simulink model "pmsm_id_bench"  (R2024b)
settings: Solver=ode4  StartTime=0.0  StopTime=bench.StopTime  FixedStep=bench.SolverStep  RelTol=1e-3
model workspace (MAT data in the model file):
  bench.Rs = 0.7
  bench.Ld = 0.004
  bench.Lq = 0.006
  bench.Flux = 0.03
  bench.VoltageDrop = 0.35
  bench.ResistanceDrop = 0.03
  bench.ZeroCurrent = 0.15
  bench.Phase = 0
  bench.StopTime = 0.6
  bench.SolverStep = 1e-05
  bench.SamplePeriod = 0.0001
  bench.InitialDCurrent = 0
  bench.InitialQCurrent = 0
  bench.DVoltageBias = 1.2
  bench.DVoltageAmplitude = [0.8 0.35]
  bench.DVoltageFrequency = [31 9]
  bench.QVoltageBias = 5
  bench.QVoltageAmplitude = [1.1 0.6]
  bench.QVoltageFrequency = [17 4]
  bench.SpeedBias = 160
  bench.SpeedAmplitude = 40
  bench.SpeedFrequency = 3
values from neighbouring files (symbols this model uses):
  bench = struct('Rs',0.7,'Ld',0.004,'Lq',0.006,'Flux',0.03,      'VoltageDrop',0.35,'ResistanceDrop',0.03,'ZeroCurrent',0.15,      'Phase',0,'StopTime',0.6,'SolverStep',1e-5,'SamplePeriod',1e-4,      'InitialDCurrent',0,'InitialQCurrent',0,      'DVoltageBias',1.2,'DVoltageAmplitude',[0.8,0.35],      'DVoltageFrequency',[31,9],'QVoltageBias',5,      'QVoltageAmplitude',[1.1,0.6],'QVoltageFrequency',[17,4], ...(+61 chars)    [pmsm_bench_defaults.m]    (also in pmsm_mechanical_defaults.m = struct('J',0.002,'B',0.001,'Tc',0.02,'FrictionSpeed',0.2,   ; pmsm_run_mechanical_benchmark.m = pmsm_mechanical_defaults(); pmsm_run_simulink_benchmark.m = pmsm_bench_defaults())
settings Model: Creator=lxy  LastModifiedBy=lxy
settings DataIOCC: SignalLogging=off

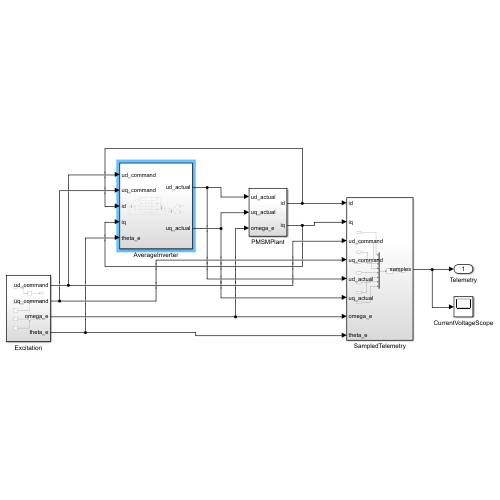
[thumbnail: Simulink's stored preview of the top-level diagram]
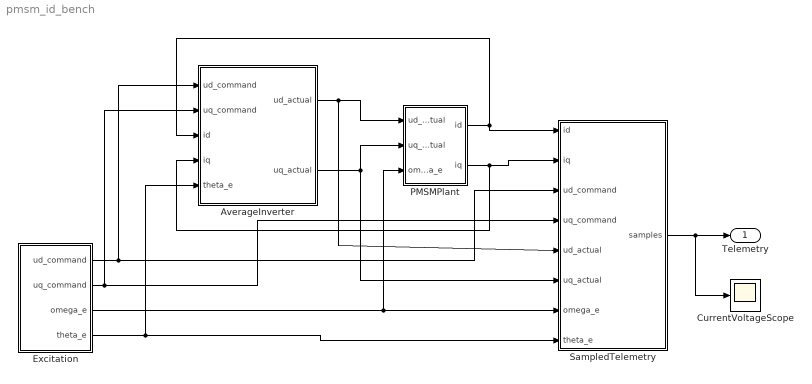
== system pmsm_id_bench ==
  AverageInverter : Subsystem
  CurrentVoltageScope : Scope
  Excitation : Subsystem
  PMSMPlant : Subsystem
  SampledTelemetry : Subsystem
  Telemetry : Outport
  wires:
  Excitation/1(ud_command) -> SampledTelemetry/3(ud_command), AverageInverter/1(ud_command)
  Excitation/2(uq_command) -> SampledTelemetry/4(uq_command), AverageInverter/2(uq_command)
  Excitation/4(theta_e) -> SampledTelemetry/8(theta_e), AverageInverter/5(theta_e)
  Excitation/3(omega_e) -> SampledTelemetry/7(omega_e), PMSMPlant/3(omega_e)
  AverageInverter/1(ud_actual) -> SampledTelemetry/5(ud_actual), PMSMPlant/1(ud_actual)
  AverageInverter/2(uq_actual) -> SampledTelemetry/6(uq_actual), PMSMPlant/2(uq_actual)
  PMSMPlant/1(id) -> SampledTelemetry/1(id), AverageInverter/3(id)
  PMSMPlant/2(iq) -> SampledTelemetry/2(iq), AverageInverter/4(iq)
  SampledTelemetry/1(samples) -> Telemetry/1, CurrentVoltageScope/1

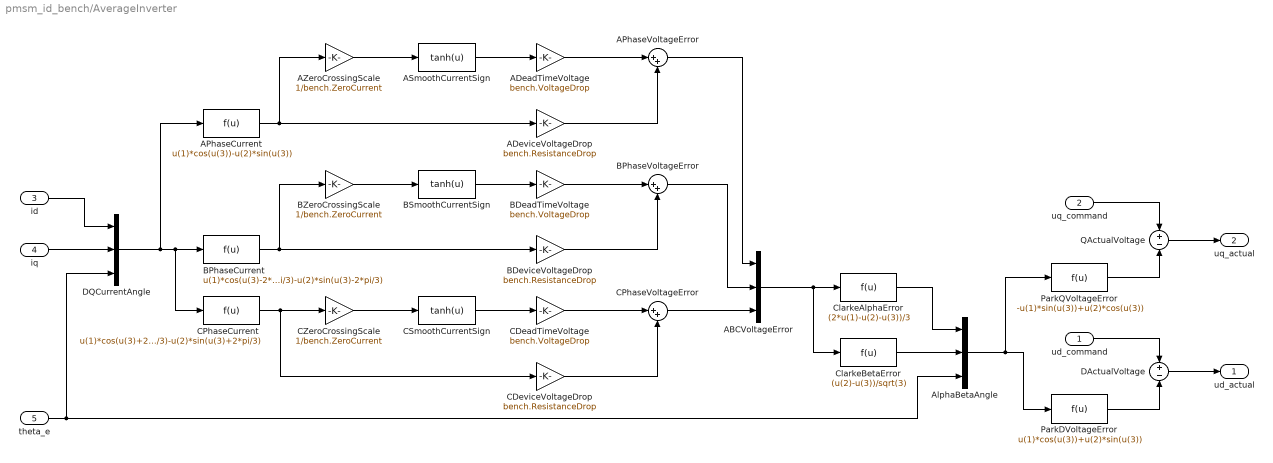
== system pmsm_id_bench/AverageInverter ==
  ud_command : Inport
  uq_command : Inport  Port=2
  id : Inport  Port=3
  iq : Inport  Port=4
  theta_e : Inport  Port=5
  ABCVoltageError : Mux  Inputs=3
  ADeadTimeVoltage : Gain  Gain=bench.VoltageDrop
  ADeviceVoltageDrop : Gain  Gain=bench.ResistanceDrop
  APhaseCurrent : Fcn  Expr=u(1)*cos(u(3))-u(2)*sin(u(3))
  APhaseVoltageError : Sum  Inputs=|++
  ASmoothCurrentSign : Fcn  Expr=tanh(u)
  AZeroCrossingScale : Gain  Gain=1/bench.ZeroCurrent
  AlphaBetaAngle : Mux  Inputs=3
  BDeadTimeVoltage : Gain  Gain=bench.VoltageDrop
  BDeviceVoltageDrop : Gain  Gain=bench.ResistanceDrop
  BPhaseCurrent : Fcn  Expr=u(1)*cos(u(3)-2*pi/3)-u(2)*sin(u(3)-2*pi/3)
  BPhaseVoltageError : Sum  Inputs=|++
  BSmoothCurrentSign : Fcn  Expr=tanh(u)
  BZeroCrossingScale : Gain  Gain=1/bench.ZeroCurrent
  CDeadTimeVoltage : Gain  Gain=bench.VoltageDrop
  CDeviceVoltageDrop : Gain  Gain=bench.ResistanceDrop
  CPhaseCurrent : Fcn  Expr=u(1)*cos(u(3)+2*pi/3)-u(2)*sin(u(3)+2*pi/3)
  CPhaseVoltageError : Sum  Inputs=|++
  CSmoothCurrentSign : Fcn  Expr=tanh(u)
  CZeroCrossingScale : Gain  Gain=1/bench.ZeroCurrent
  ClarkeAlphaError : Fcn  Expr=(2*u(1)-u(2)-u(3))/3
  ClarkeBetaError : Fcn  Expr=(u(2)-u(3))/sqrt(3)
  DActualVoltage : Sum  Inputs=+-
  DQCurrentAngle : Mux  Inputs=3
  ParkDVoltageError : Fcn  Expr=u(1)*cos(u(3))+u(2)*sin(u(3))
  ParkQVoltageError : Fcn  Expr=-u(1)*sin(u(3))+u(2)*cos(u(3))
  QActualVoltage : Sum  Inputs=+-
  ud_actual : Outport
  uq_actual : Outport  Port=2
  wires:
  QActualVoltage/1 -> uq_actual/1
  DActualVoltage/1 -> ud_actual/1
  ParkQVoltageError/1 -> QActualVoltage/2
  uq_command/1 -> QActualVoltage/1
  ParkDVoltageError/1 -> DActualVoltage/2
  ud_command/1 -> DActualVoltage/1
  AlphaBetaAngle/1 -> ParkDVoltageError/1, ParkQVoltageError/1
  ClarkeBetaError/1 -> AlphaBetaAngle/2
  ClarkeAlphaError/1 -> AlphaBetaAngle/1
  ABCVoltageError/1 -> ClarkeAlphaError/1, ClarkeBetaError/1
  CPhaseVoltageError/1 -> ABCVoltageError/3
  BPhaseVoltageError/1 -> ABCVoltageError/2
  APhaseVoltageError/1 -> ABCVoltageError/1
  CDeviceVoltageDrop/1 -> CPhaseVoltageError/2
  CDeadTimeVoltage/1 -> CPhaseVoltageError/1
  CSmoothCurrentSign/1 -> CDeadTimeVoltage/1
  CZeroCrossingScale/1 -> CSmoothCurrentSign/1
  CPhaseCurrent/1 -> CZeroCrossingScale/1, CDeviceVoltageDrop/1
  BDeviceVoltageDrop/1 -> BPhaseVoltageError/2
  BDeadTimeVoltage/1 -> BPhaseVoltageError/1
  BSmoothCurrentSign/1 -> BDeadTimeVoltage/1
  BZeroCrossingScale/1 -> BSmoothCurrentSign/1
  BPhaseCurrent/1 -> BZeroCrossingScale/1, BDeviceVoltageDrop/1
  ADeviceVoltageDrop/1 -> APhaseVoltageError/2
  ADeadTimeVoltage/1 -> APhaseVoltageError/1
  ASmoothCurrentSign/1 -> ADeadTimeVoltage/1
  AZeroCrossingScale/1 -> ASmoothCurrentSign/1
  APhaseCurrent/1 -> AZeroCrossingScale/1, ADeviceVoltageDrop/1
  DQCurrentAngle/1 -> BPhaseCurrent/1, CPhaseCurrent/1, APhaseCurrent/1
  theta_e/1 -> DQCurrentAngle/3, AlphaBetaAngle/3
  iq/1 -> DQCurrentAngle/2
  id/1 -> DQCurrentAngle/1

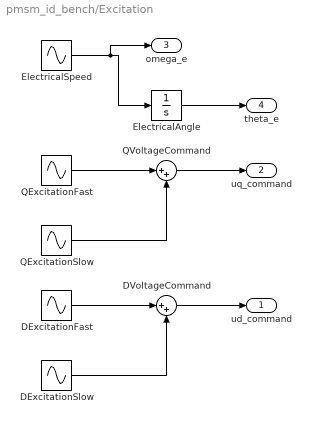
== system pmsm_id_bench/Excitation ==
  DExcitationFast : Sin  Amplitude=bench.DVoltageAmplitude(1)  Frequency=2*pi*bench.DVoltageFrequency(1)  Phase=bench.Phase  SampleTime=0
  DExcitationSlow : Sin  Amplitude=bench.DVoltageAmplitude(2)  Bias=bench.DVoltageBias  Frequency=2*pi*bench.DVoltageFrequency(2)  SampleTime=0
  DVoltageCommand : Sum  Inputs=|++
  ElectricalAngle : Integrator
  ElectricalSpeed : Sin  Amplitude=bench.SpeedAmplitude  Bias=bench.SpeedBias  Frequency=2*pi*bench.SpeedFrequency  Phase=bench.Phase  SampleTime=0
  QExcitationFast : Sin  Amplitude=bench.QVoltageAmplitude(1)  Frequency=2*pi*bench.QVoltageFrequency(1)  Phase=pi/2+bench.Phase  SampleTime=0
  QExcitationSlow : Sin  Amplitude=bench.QVoltageAmplitude(2)  Bias=bench.QVoltageBias  Frequency=2*pi*bench.QVoltageFrequency(2)  SampleTime=0
  QVoltageCommand : Sum  Inputs=|++
  ud_command : Outport
  uq_command : Outport  Port=2
  omega_e : Outport  Port=3
  theta_e : Outport  Port=4
  wires:
  ElectricalAngle/1 -> theta_e/1
  ElectricalSpeed/1 -> omega_e/1, ElectricalAngle/1
  QVoltageCommand/1 -> uq_command/1
  QExcitationSlow/1 -> QVoltageCommand/2
  QExcitationFast/1 -> QVoltageCommand/1
  DVoltageCommand/1 -> ud_command/1
  DExcitationSlow/1 -> DVoltageCommand/2
  DExcitationFast/1 -> DVoltageCommand/1

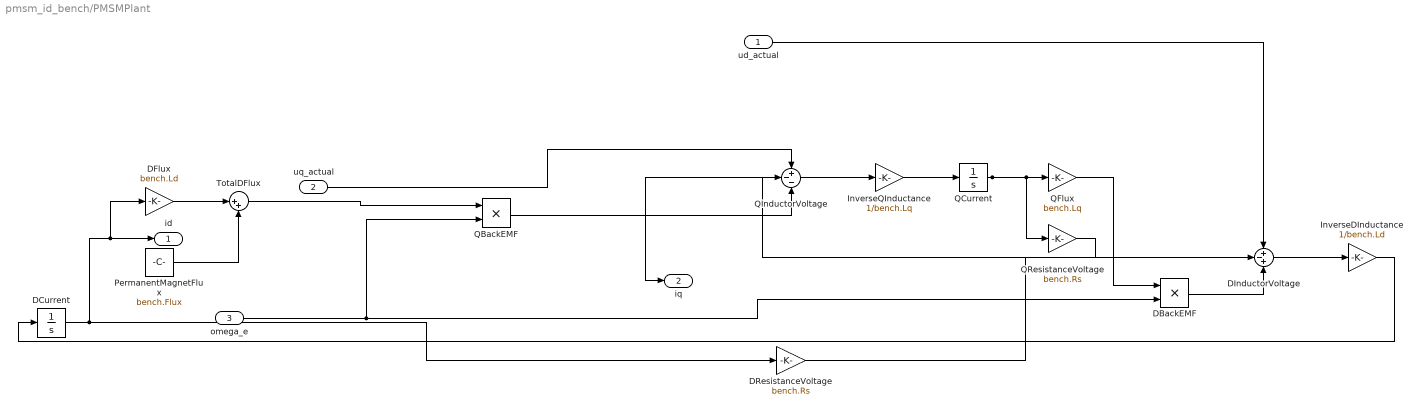
== system pmsm_id_bench/PMSMPlant ==
  ud_actual : Inport
  uq_actual : Inport  Port=2
  omega_e : Inport  Port=3
  DBackEMF : Product  Inputs=**
  DCurrent : Integrator  InitialCondition=bench.InitialDCurrent
  DFlux : Gain  Gain=bench.Ld
  DInductorVoltage : Sum  Inputs=+-+
  DResistanceVoltage : Gain  Gain=bench.Rs
  InverseDInductance : Gain  Gain=1/bench.Ld
  InverseQInductance : Gain  Gain=1/bench.Lq
  PermanentMagnetFlux : Constant  Value=bench.Flux
  QBackEMF : Product  Inputs=**
  QCurrent : Integrator  InitialCondition=bench.InitialQCurrent
  QFlux : Gain  Gain=bench.Lq
  QInductorVoltage : Sum  Inputs=+--
  QResistanceVoltage : Gain  Gain=bench.Rs
  TotalDFlux : Sum  Inputs=|++
  id : Outport
  iq : Outport  Port=2
  wires:
  InverseQInductance/1 -> QCurrent/1
  InverseDInductance/1 -> DCurrent/1
  QInductorVoltage/1 -> InverseQInductance/1
  DInductorVoltage/1 -> InverseDInductance/1
  QBackEMF/1 -> QInductorVoltage/3
  QResistanceVoltage/1 -> QInductorVoltage/2
  uq_actual/1 -> QInductorVoltage/1
  DBackEMF/1 -> DInductorVoltage/3
  DResistanceVoltage/1 -> DInductorVoltage/2
  ud_actual/1 -> DInductorVoltage/1
  QFlux/1 -> DBackEMF/1
  omega_e/1 -> QBackEMF/2, DBackEMF/2
  TotalDFlux/1 -> QBackEMF/1
  PermanentMagnetFlux/1 -> TotalDFlux/2
  DFlux/1 -> TotalDFlux/1
  QCurrent/1 -> QResistanceVoltage/1, QFlux/1, iq/1
  DCurrent/1 -> id/1, DFlux/1, DResistanceVoltage/1

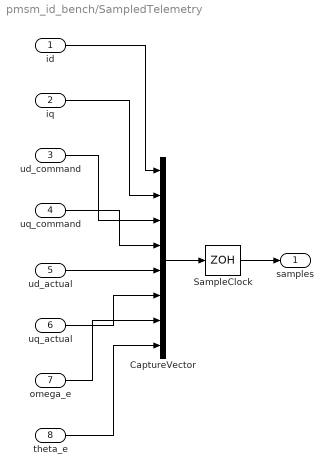
== system pmsm_id_bench/SampledTelemetry ==
  id : Inport
  iq : Inport  Port=2
  ud_command : Inport  Port=3
  uq_command : Inport  Port=4
  ud_actual : Inport  Port=5
  uq_actual : Inport  Port=6
  omega_e : Inport  Port=7
  theta_e : Inport  Port=8
  CaptureVector : Mux  Inputs=8
  SampleClock : ZeroOrderHold  SampleTime=bench.SamplePeriod
  samples : Outport
  wires:
  theta_e/1 -> CaptureVector/8
  omega_e/1 -> CaptureVector/7
  uq_actual/1 -> CaptureVector/6
  ud_actual/1 -> CaptureVector/5
  uq_command/1 -> CaptureVector/4
  ud_command/1 -> CaptureVector/3
  iq/1 -> CaptureVector/2
  id/1 -> CaptureVector/1
  SampleClock/1 -> samples/1
  CaptureVector/1 -> SampleClock/1
